simulink model "my_cascade_ramp116_rt"  (R2024a)
settings: Solver=ode3  StartTime=0.0  StopTime=40  FixedStep=0.003  RelTol=1e-3  EnableMultiTasking=on
PreLoadFcn:
  | load('C:\Users\hp\Desktop\group_22\group22_sensor.mat');
undefined symbols (not defined in the file or in its folder): DiscIntNeverNeededParam
libraries: simulink x1
settings Model: SimulationMode=external  Creator=kha  LastModifiedBy=hp
settings SolverCC: AlgebraicLoopSolver=TrustRegion
settings DataIOCC: LimitDataPoints=on  SaveFormat=Array  SignalLoggingSaveFormat=ModelDataLogs  ReturnWorkspaceOutputs=off
settings OptimizationCC: ExpressionDepthLimit=2147483647  InitFltsAndDblsToZero=on  LifeSpan=inf
settings DebuggingCC: SaveWithParameterizedLinksMsg=none  UnderspecifiedInitializationDetection=Classic  MergeDetectMultiDrivingBlocksExec=none  SolverPrmCheckMsg=warning  FcnCallInpInsideContextMsg=warning  UnconnectedInputMsg=warning  UnconnectedOutputMsg=warning  UnconnectedLineMsg=warning  StateNameClashWarn=warning  SFUnexpectedBacktrackingDiag=warning  SFNoUnconditionalDefaultTransitionDiag=warning  SFExecutionAtInitializationDiag=none  ArithmeticOperatorsInVariantConditions=warning
settings HardwareCC: ProdBitPerPointer=32  ProdBitPerSizeT=32  ProdBitPerPtrDiffT=32  ProdLargestAtomicFloat=None  ProdIntDivRoundTo=Undefined  ProdEndianess=Unspecified  ProdWordSize=32  ProdHWDeviceType=32-bit Generic
settings ModelReferenceCC: EnableRefExpFcnMdlSchedulingChecks=on  PropagateSignalLabelsOutOfModel=off
settings SFSimCC: SimUseLocalCustomCode=off  CustomCodeUndefinedFunction=UseInterfaceOnly
settings RTWCC: Description=MLS1EM-RTDAC/USB2 (Visual C/C++)  SystemTargetFile=mls1em_rtcon_usb2.tlc  TemplateMakefile=MLS1EM_RTCON_VC_USB2_x64.tmf  RTWUseLocalCustomCode=off  GPUComputeCapability=3.5  DLArmComputeVersion=19.05
settings CodeAppCC: StateflowObjectComments=on
settings STFCustomTargetCC: TargetLangStandard=C89/C90 (ANSI)  ModelReferenceCompliant=off  CombineOutputUpdateFcns=on  MatFileLogging=on  GRTInterface=off  UseToolchainInfoCompliant=off  SystemTargetFile=mls1em_rtcon_usb2.tlc
settings GRTTargetCC: TargetLangStandard=C89/C90 (ANSI)  ModelReferenceCompliant=off  ParMdlRefBuildCompliant=off  CompOptLevelCompliant=off  ConcurrentExecutionCompliant=off  CPPClassGenCompliant=off  UseToolchainInfoCompliant=off  ExtMode=on  ExtModeMexFile=rtcon_ext_comm
settings ConfigComp: CovMetricSettings=dw  CovSaveCumulativeToWorkspaceVar=on  CovSaveSingleToWorkspaceVar=on  CovExternalEMLEnable=off  CovSFcnEnable=off

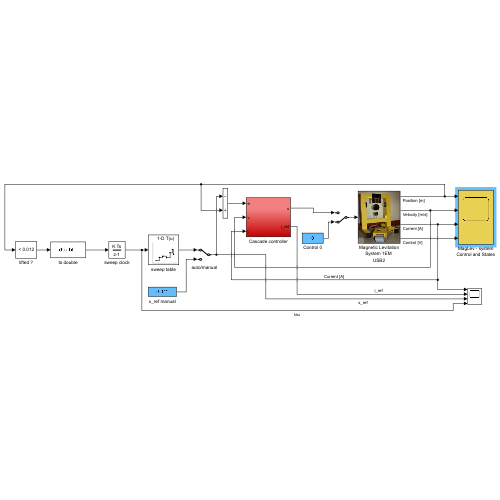
[thumbnail: Simulink's stored preview of the top-level diagram]
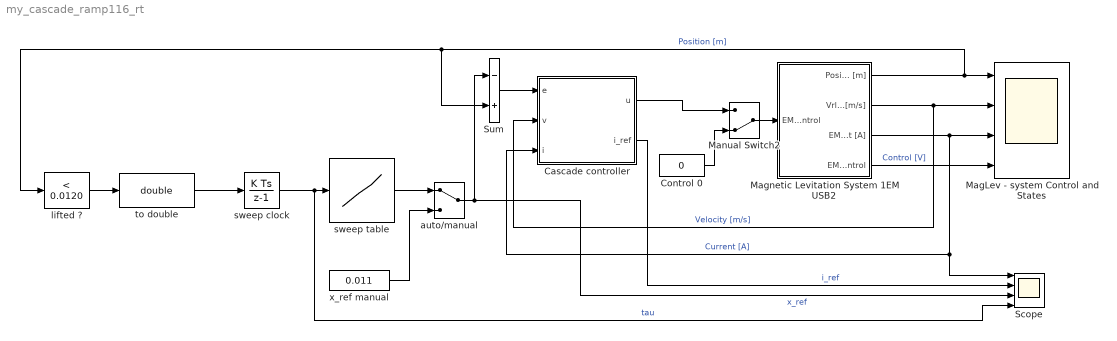
== system my_cascade_ramp116_rt ==
  Cascade controller : Subsystem
  Control 0 : Constant  Value=0
  MagLev - system Control and States : Scope  NumInputPorts=4
  Magnetic Levitation System 1EM USB2 : Subsystem  mask(Magnetic Levitation MLS1EM - System){RTDACUSB2IDX=-1, T0=0.003}
      mask prompts: RTDACUSB2IDX "RT-DAC/USB2 Board Idx (-1) for auto detect"; T0 "Sample time [s]"
      mask help:
      | MagLev MLS2EM - System connection for the real-time operating mode, RT-DAC/USB2 interface
      | (c) InTeCo 2015
      mask Display: image(imread('mls1em_usb2.tiff'));
  Manual Switch2 : ManualSwitch  CurrentSetting=0
  Scope : Scope  NumInputPorts=4
  Sum : Sum  Inputs=-+  InputSameDT=on  SaturateOnIntegerOverflow=on  OutDataTypeStr=Inherit: Same as first input
  auto/manual : ManualSwitch
  lifted ? : simulink/Logic and Bit Operations/Compare To Constant  relop=<  const=0.0120  OutDataTypeStr=boolean
  sweep clock : DiscreteIntegrator  SampleTime=0.003  ICPrevOutput=DiscIntNeverNeededParam  ICPrevScaledInput=DiscIntNeverNeededParam
  sweep table : Lookup_n-D  NumberOfTableDimensions=1  BreakpointsForDimension1=[0 5 10 15.5 21 26]  Table=[11 10.5 10.5 11.6 10.5 10.5]*1e-3  InterpMethod=Flat  InternalRulePriority=Speed  RndMeth=Simplest
  to double : DataTypeConversion  OutDataTypeStr=double  SaturateOnIntegerOverflow=off  RndMeth=Floor
  x_ref manual : Constant  Value=0.011
  wires:
  Control 0/1 -> Manual Switch2/2
  Magnetic Levitation System 1EM USB2/1(Position [m]) -> lifted ?/1, Sum/2, MagLev - system Control and States/1  "Position [m]"
  Magnetic Levitation System 1EM USB2/2(Vrlocity [m/s]) -> Cascade controller/2(v), MagLev - system Control and States/2  "Velocity [m/s]"
  Magnetic Levitation System 1EM USB2/3(EM1 Current [A]) -> Scope/1, Cascade controller/3(i), MagLev - system Control and States/3  "Current [A]"
  Magnetic Levitation System 1EM USB2/4(EM1 control) -> MagLev - system Control and States/4  "Control [V]"
  Manual Switch2/1 -> Magnetic Levitation System 1EM USB2/1(EM1 Control)
  Sum/1 -> Cascade controller/1(e)
  Cascade controller/1(u) -> Manual Switch2/1
  Cascade controller/2(i_ref) -> Scope/2  "i_ref"
  lifted ?/1 -> to double/1
  to double/1 -> sweep clock/1
  sweep clock/1 -> Scope/4, sweep table/1  "tau"
  sweep table/1 -> auto/manual/1
  x_ref manual/1 -> auto/manual/2
  auto/manual/1 -> Scope/3, Sum/1  "x_ref"

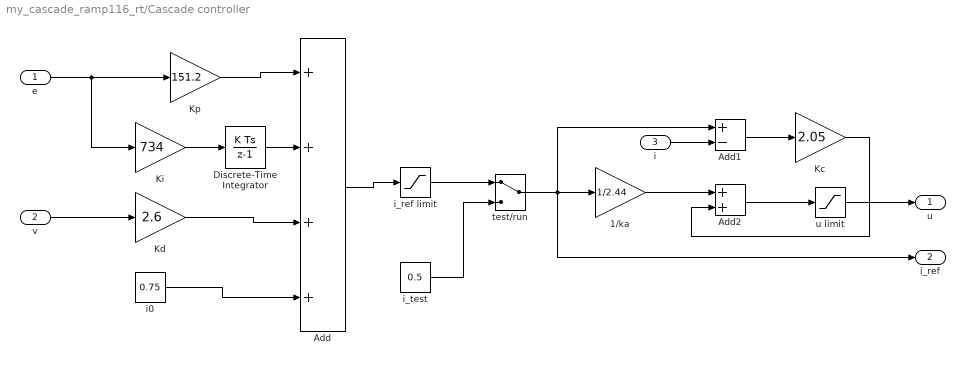
== system my_cascade_ramp116_rt/Cascade controller ==
  e : Inport
  v : Inport  Port=2
  i : Inport  Port=3
  1/ka : Gain  Gain=1/2.44
  Add : Sum  Inputs=++++
  Add1 : Sum  Inputs=+-
  Add2 : Sum
  Discrete-Time Integrator : DiscreteIntegrator  SampleTime=0.003  LimitOutput=on  UpperSaturationLimit=0.3  LowerSaturationLimit=-0.3  ICPrevOutput=DiscIntNeverNeededParam  ICPrevScaledInput=DiscIntNeverNeededParam
  Kc : Gain  Gain=2.05
  Kd : Gain  Gain=2.6
  Ki : Gain  Gain=734
  Kp : Gain  Gain=151.2
  i0 : Constant  Value=0.75
  i_ref limit : Saturate  UpperLimit=2.0  LowerLimit=0
      settings: AttributesFormatString=|
      | UL: %<UpperLimit>
      | LL: %<LowerLimit>
  i_test : Constant  Value=0.5
  test/run : ManualSwitch
  u limit : Saturate  UpperLimit=0.9  LowerLimit=0
      settings: AttributesFormatString=|
      | UL: %<UpperLimit>
      | LL: %<LowerLimit>
  u : Outport
  i_ref : Outport  Port=2
  wires:
  e/1 -> Kp/1, Ki/1
  Kp/1 -> Add/1
  Ki/1 -> Discrete-Time Integrator/1
  Discrete-Time Integrator/1 -> Add/2
  Kd/1 -> Add/3
  v/1 -> Kd/1
  i0/1 -> Add/4
  Add/1 -> i_ref limit/1
  i_ref limit/1 -> test/run/1
  i_test/1 -> test/run/2
  test/run/1 -> i_ref/1, 1/ka/1, Add1/1
  1/ka/1 -> Add2/1
  i/1 -> Add1/2
  Add1/1 -> Kc/1
  Kc/1 -> Add2/2
  Add2/1 -> u limit/1
  u limit/1 -> u/1

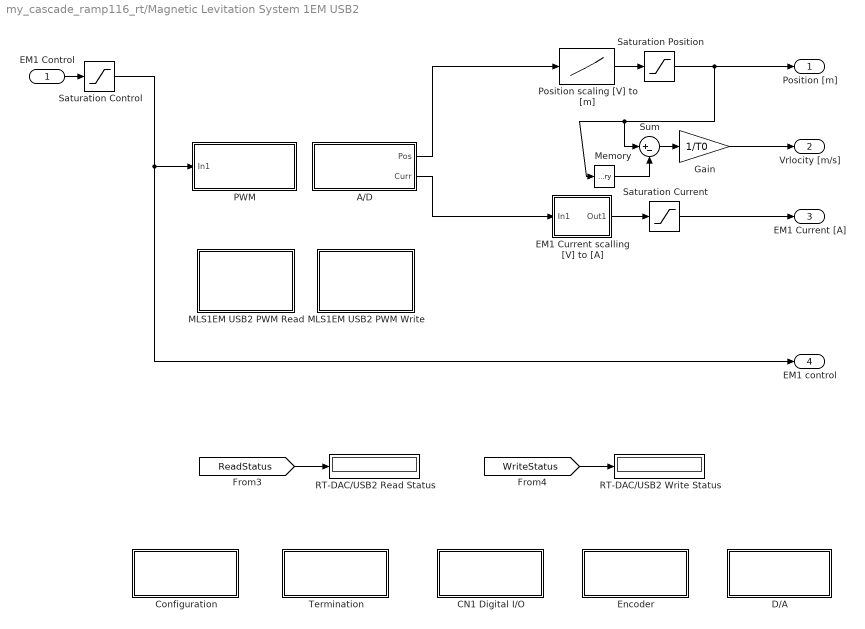
== system my_cascade_ramp116_rt/Magnetic Levitation System 1EM USB2 ==
  EM1 Control : Inport
  A/D : Subsystem
      mask Display: disp('A / D')
  CN1 Digital I/O : Subsystem
      mask Display: disp('CN1 Digital I/O')
  Configuration : Subsystem
      mask Display: disp('CONFIGURATION')
  D/A : Subsystem
      mask Display: disp('D / A')
  EM1 Current scalling [V] to [A] : Subsystem
      mask Display: plot([0    0.5000    1.0000    1.5000    2.0000    2.5000], [-0.0317    0.4951    1.0302    1.5738    2.1258    2.6863]);
  Encoder : Subsystem
      mask Display: disp('Encoder')
  Gain : Gain  Gain=1/T0
  MLS1EM USB2 PWM Read : Subsystem
      mask Display: disp( 'RT-DAC/USB2' )
  MLS1EM USB2 PWM Write : Subsystem
      mask Display: disp( 'RT-DAC/USB2')
  Memory : Memory
  PWM : Subsystem
      mask Display: disp('PWM')
  Position scaling [V] to [m] : Lookup  InputValues=SensorData.Sensor_V(end:-1:1)  Table=SensorData.Distance_m(end:-1:1)
  RT-DAC/USB2 Read Status : Display
  RT-DAC/USB2 Write Status : Display
  Saturation Control : Saturate  UpperLimit=5  LowerLimit=0
  Saturation Current : Saturate  UpperLimit=30  LowerLimit=-30
  Saturation Position : Saturate  UpperLimit=0.02  LowerLimit=0
  Sum : Sum  Inputs=|+-
  Termination : Subsystem
      mask Display: disp('CONFIGURATION')
  Position [m] : Outport  VectorParamsAs1DForOutWhenUnconnected=off
  Vrlocity [m/s] : Outport  Port=2  VectorParamsAs1DForOutWhenUnconnected=off
  EM1 Current [A] : Outport  Port=3  VectorParamsAs1DForOutWhenUnconnected=off
  EM1 control : Outport  Port=4  VectorParamsAs1DForOutWhenUnconnected=off
  wires:
  EM1 Control/1 -> Saturation Control/1
  Saturation Position/1 -> Position [m]/1, Sum/1, Memory/1
  Gain/1 -> Vrlocity [m/s]/1
  Saturation Control/1 -> PWM/1(In1), EM1 control/1
  Memory/1 -> Sum/2
  Position scaling [V] to [m]/1 -> Saturation Position/1
  Sum/1 -> Gain/1
  EM1 Current scalling [V] to [A]/1(Out1) -> Saturation Current/1
  [ReadStatus] -> RT-DAC/USB2 Read Status/1
  [WriteStatus] -> RT-DAC/USB2 Write Status/1
  A/D/1(Pos) -> Position scaling [V] to [m]/1
  A/D/2(Curr) -> EM1 Current scalling [V] to [A]/1(In1)
  Saturation Current/1 -> EM1 Current [A]/1

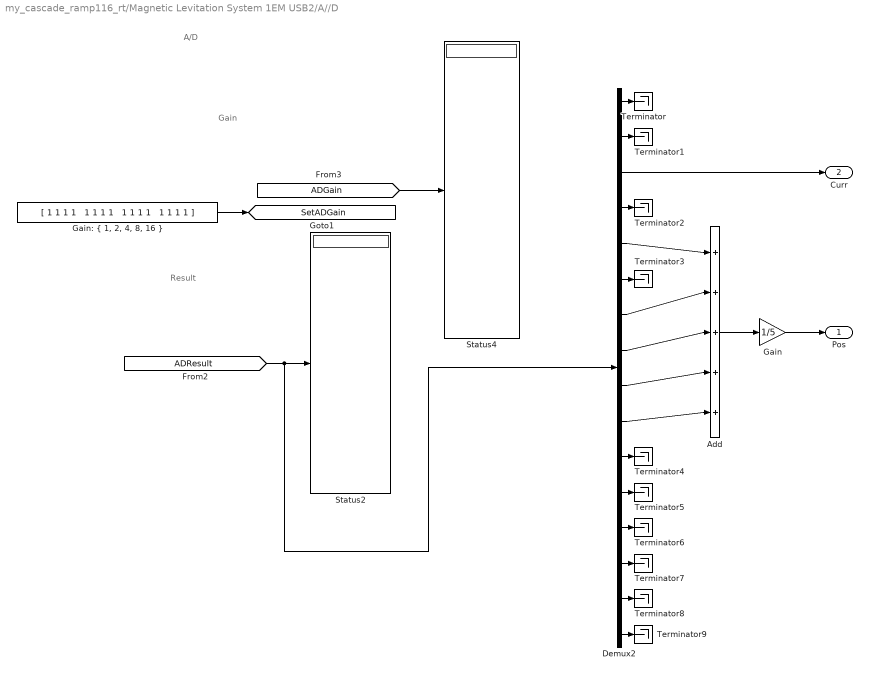
== system my_cascade_ramp116_rt/Magnetic Levitation System 1EM USB2/A//D ==
  note: A/D
  note: Gain
  note: Result
  Add : Sum  Inputs=+|++++
  Demux2 : Demux  Outputs=16
      settings: DisplayOption=none
  Gain : Gain  Gain=1/5
  "Gain: { 1, 2, 4, 8, 16 }" : Constant  Value="[ 1 1 1 1   1 1 1 1   1 1 1 1   1 1 1 1 ]"
  Status2 : Display
  Status4 : Display
  Terminator{,1..9} (10 alike) : Terminator
  Pos : Outport  VectorParamsAs1DForOutWhenUnconnected=off
  Curr : Outport  Port=2  VectorParamsAs1DForOutWhenUnconnected=off
  tag scope: SetADGain=global
  wires:
  [ADResult] -> Demux2/1, Status2/1
  [ADGain] -> Status4/1
  "Gain: { 1, 2, 4, 8, 16 }"/1 -> [SetADGain]
  Add/1 -> Gain/1
  Gain/1 -> Pos/1
  Demux2/3 -> Curr/1
  Demux2/5 -> Add/1
  Demux2/7 -> Add/2
  Demux2/8 -> Add/3
  Demux2/9 -> Add/4
  Demux2/10 -> Add/5
  Demux2/1 -> Terminator/1
  Demux2/2 -> Terminator1/1
  Demux2/4 -> Terminator2/1
  Demux2/6 -> Terminator3/1
  Demux2/11 -> Terminator4/1
  Demux2/12 -> Terminator5/1
  Demux2/13 -> Terminator6/1
  Demux2/14 -> Terminator7/1
  Demux2/15 -> Terminator8/1
  Demux2/16 -> Terminator9/1

== system my_cascade_ramp116_rt/Magnetic Levitation System 1EM USB2/CN1 Digital I//O ==
  note: Digital I/Os
  note: Pin mode
  note: Direction
  note: Output
  note: Input
  Data Type Conversion1 : DataTypeConversion  OutDataTypeStr=uint32  SaturateOnIntegerOverflow=off  RndMeth=Floor
  Data Type Conversion2 : DataTypeConversion  OutDataTypeStr=int32  SaturateOnIntegerOverflow=off  RndMeth=Floor
  Data Type Conversion3 : DataTypeConversion  OutDataTypeStr=uint32  SaturateOnIntegerOverflow=off  RndMeth=Floor
  Data Type Conversion4 : DataTypeConversion  OutDataTypeStr=int32  SaturateOnIntegerOverflow=off  RndMeth=Floor
  Status{1..4} (4 alike) : Display
      settings: Format=hex (Stored Integer)
  Subsystem : Subsystem
      mask Display: disp( 'CN1 Direction' )
  Subsystem1 : Subsystem
      mask Display: disp( 'CN1 Output' )
  Subsystem2 : Subsystem
      mask Display: disp( 'CN1 Pin Mode' )
  wires:
  Data Type Conversion1/1 -> Status1/1
  Data Type Conversion2/1 -> Status3/1
  [CN1Direction] -> Data Type Conversion1/1
  [CN1PinMode] -> Data Type Conversion2/1
  Data Type Conversion3/1 -> Status2/1
  Data Type Conversion4/1 -> Status4/1
  [CN1Output] -> Data Type Conversion4/1
  [CN1Input] -> Data Type Conversion3/1

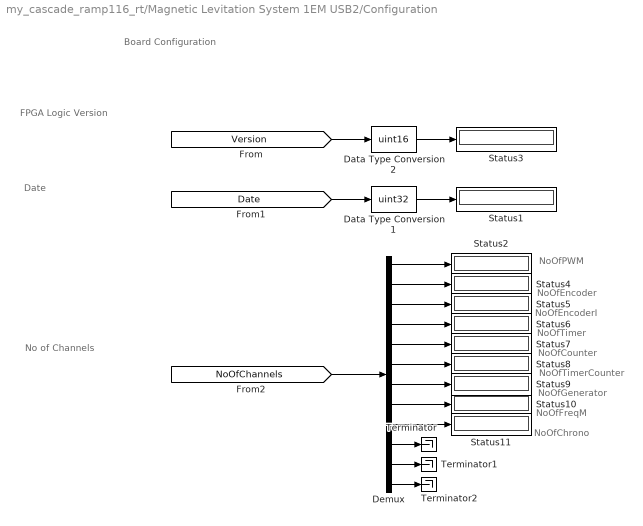
== system my_cascade_ramp116_rt/Magnetic Levitation System 1EM USB2/Configuration ==
  note: NoOfPWM
  note: NoOfEncoder
  note: NoOfEncoderI
  note: NoOfTimer
  note: NoOfCounter
  note: NoOfTimerCounter
  note: NoOfGenerator
  note: NoOfFreqM
  note: NoOfChrono
  note: Board Configuration
  note: FPGA Logic
      | Version
  note: Date
  note: No of
      | Channels
  Data Type Conversion1 : DataTypeConversion  OutDataTypeStr=uint32  SaturateOnIntegerOverflow=off  RndMeth=Floor
  Data Type Conversion2 : DataTypeConversion  OutDataTypeStr=uint16  SaturateOnIntegerOverflow=off  RndMeth=Floor
  Demux : Demux  Outputs=12
  Status{1..11} (11 alike) : Display
      Status1 settings: Format=hex (Stored Integer)
      Status3 settings: Format=hex (Stored Integer)
  Terminator : Terminator
  Terminator1 : Terminator
  Terminator2 : Terminator
  wires:
  [Version] -> Data Type Conversion2/1
  [Date] -> Data Type Conversion1/1
  Data Type Conversion2/1 -> Status3/1
  Data Type Conversion1/1 -> Status1/1
  [NoOfChannels] -> Demux/1
  Demux/1 -> Status2/1
  Demux/2 -> Status4/1
  Demux/3 -> Status5/1
  Demux/4 -> Status6/1
  Demux/5 -> Status7/1
  Demux/6 -> Status8/1
  Demux/7 -> Status9/1
  Demux/8 -> Status10/1
  Demux/9 -> Status11/1
  Demux/10 -> Terminator/1
  Demux/11 -> Terminator1/1
  Demux/12 -> Terminator2/1

== system my_cascade_ramp116_rt/Magnetic Levitation System 1EM USB2/D//A ==
  note: D/A
  note: D/A outputs range: -10.0 - +10.0
  D/A {0..3} (4 alike) : Constant  Value=0
  Mux1 : Mux
  Status4 : Display
  tag scope: SetDA=global
  wires:
  Mux1/1 -> [SetDA]
  [DA] -> Status4/1
  D/A 1/1 -> Mux1/2
  D/A 2/1 -> Mux1/3
  D/A 3/1 -> Mux1/4
  D/A 0/1 -> Mux1/1

== system my_cascade_ramp116_rt/Magnetic Levitation System 1EM USB2/EM1 Current scalling [V] to [A] ==
  In1 : Inport
  Fcn : Fcn  Expr=0.598941443808775*u(1)-0.017342099593970
  Out1 : Outport  VectorParamsAs1DForOutWhenUnconnected=off
  wires:
  In1/1 -> Fcn/1
  Fcn/1 -> Out1/1

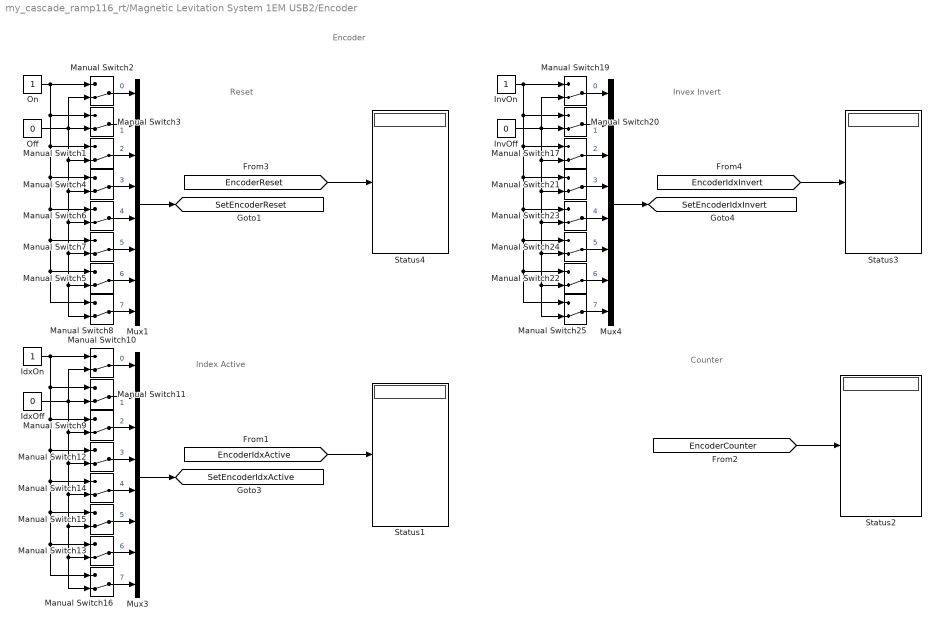
== system my_cascade_ramp116_rt/Magnetic Levitation System 1EM USB2/Encoder ==
  note: Counter
  note: Reset
  note: Encoder
  note: Index Active
  note: Invex Invert
  IdxOff : Constant  Value=0
  IdxOn : Constant
  InvOff : Constant  Value=0
  InvOn : Constant
  Manual Switch{1..17,19..25} (24 alike) : ManualSwitch  CurrentSetting=0
  Mux1 : Mux  Inputs=8
  Mux3 : Mux  Inputs=8
  Mux4 : Mux  Inputs=8
  Off : Constant  Value=0
  On : Constant
  Status{1..4} (4 alike) : Display
  tag scope: SetEncoderIdxActive=global, SetEncoderIdxInvert=global, SetEncoderReset=global
  wires:
  Manual Switch8/1 -> Mux1/8  "7"
  Manual Switch5/1 -> Mux1/7  "6"
  Manual Switch1/1 -> Mux1/3  "2"
  Manual Switch4/1 -> Mux1/4  "3"
  Manual Switch7/1 -> Mux1/6  "5"
  Manual Switch6/1 -> Mux1/5  "4"
  Manual Switch3/1 -> Mux1/2  "1"
  Manual Switch2/1 -> Mux1/1  "0"
  Off/1 -> Manual Switch8/2, Manual Switch5/2, Manual Switch7/2, Manual Switch6/2, Manual Switch4/2, Manual Switch1/2, Manual Switch2/2, Manual Switch3/2
  On/1 -> Manual Switch1/1, Manual Switch4/1, Manual Switch6/1, Manual Switch7/1, Manual Switch5/1, Manual Switch8/1, Manual Switch3/1, Manual Switch2/1
  Mux1/1 -> [SetEncoderReset]
  [EncoderReset] -> Status4/1
  [EncoderCounter] -> Status2/1
  Manual Switch16/1 -> Mux3/8  "7"
  Manual Switch13/1 -> Mux3/7  "6"
  Manual Switch9/1 -> Mux3/3  "2"
  Manual Switch12/1 -> Mux3/4  "3"
  Manual Switch15/1 -> Mux3/6  "5"
  Manual Switch14/1 -> Mux3/5  "4"
  Manual Switch11/1 -> Mux3/2  "1"
  Manual Switch10/1 -> Mux3/1  "0"
  IdxOff/1 -> Manual Switch11/2, Manual Switch10/2, Manual Switch9/2, Manual Switch12/2, Manual Switch14/2, Manual Switch15/2, Manual Switch13/2, Manual Switch16/2
  IdxOn/1 -> Manual Switch10/1, Manual Switch11/1, Manual Switch16/1, Manual Switch13/1, Manual Switch15/1, Manual Switch14/1, Manual Switch12/1, Manual Switch9/1
  Mux3/1 -> [SetEncoderIdxActive]
  [EncoderIdxActive] -> Status1/1
  Manual Switch25/1 -> Mux4/8  "7"
  Manual Switch22/1 -> Mux4/7  "6"
  Manual Switch17/1 -> Mux4/3  "2"
  Manual Switch21/1 -> Mux4/4  "3"
  Manual Switch24/1 -> Mux4/6  "5"
  Manual Switch23/1 -> Mux4/5  "4"
  Manual Switch20/1 -> Mux4/2  "1"
  Manual Switch19/1 -> Mux4/1  "0"
  InvOff/1 -> Manual Switch25/2, Manual Switch22/2, Manual Switch24/2, Manual Switch23/2, Manual Switch21/2, Manual Switch17/2, Manual Switch19/2, Manual Switch20/2
  InvOn/1 -> Manual Switch17/1, Manual Switch21/1, Manual Switch23/1, Manual Switch24/1, Manual Switch22/1, Manual Switch25/1, Manual Switch20/1, Manual Switch19/1
  Mux4/1 -> [SetEncoderIdxInvert]
  [EncoderIdxInvert] -> Status3/1

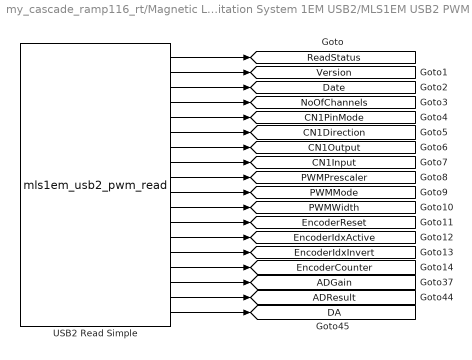
== system my_cascade_ramp116_rt/Magnetic Levitation System 1EM USB2/MLS1EM USB2 PWM Read ==
  USB2 Read Simple : S-Function  FunctionName=mls1em_usb2_pwm_read  Parameters=-1, T0  SFunctionDeploymentMode=off  EnableBusSupport=off
  tag scope: ADGain=global, ADResult=global, CN1Direction=global, CN1Input=global, CN1Output=global, CN1PinMode=global, DA=global, Date=global, EncoderCounter=global, EncoderIdxActive=global, EncoderIdxInvert=global, EncoderReset=global, NoOfChannels=global, PWMMode=global, PWMPrescaler=global, PWMWidth=global, ReadStatus=global, Version=global
  wires:
  USB2 Read Simple/18 -> [DA]
  USB2 Read Simple/17 -> [ADResult]
  USB2 Read Simple/16 -> [ADGain]
  USB2 Read Simple/1 -> [ReadStatus]
  USB2 Read Simple/2 -> [Version]
  USB2 Read Simple/3 -> [Date]
  USB2 Read Simple/4 -> [NoOfChannels]
  USB2 Read Simple/5 -> [CN1PinMode]
  USB2 Read Simple/6 -> [CN1Direction]
  USB2 Read Simple/7 -> [CN1Output]
  USB2 Read Simple/8 -> [CN1Input]
  USB2 Read Simple/9 -> [PWMPrescaler]
  USB2 Read Simple/11 -> [PWMWidth]
  USB2 Read Simple/10 -> [PWMMode]
  USB2 Read Simple/12 -> [EncoderReset]
  USB2 Read Simple/13 -> [EncoderIdxActive]
  USB2 Read Simple/14 -> [EncoderIdxInvert]
  USB2 Read Simple/15 -> [EncoderCounter]

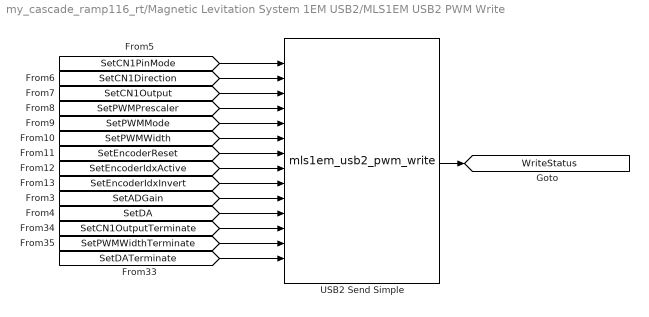
== system my_cascade_ramp116_rt/Magnetic Levitation System 1EM USB2/MLS1EM USB2 PWM Write ==
  USB2 Send Simple : S-Function  FunctionName=mls1em_usb2_pwm_write  Parameters=-1, T0  SFunctionDeploymentMode=off  EnableBusSupport=off
  tag scope: WriteStatus=global
  wires:
  [SetEncoderIdxInvert] -> USB2 Send Simple/9
  [SetPWMWidthTerminate] -> USB2 Send Simple/13
  [SetCN1OutputTerminate] -> USB2 Send Simple/12
  [SetDATerminate] -> USB2 Send Simple/14
  [SetDA] -> USB2 Send Simple/11
  [SetADGain] -> USB2 Send Simple/10
  [SetEncoderIdxActive] -> USB2 Send Simple/8
  [SetEncoderReset] -> USB2 Send Simple/7
  [SetPWMWidth] -> USB2 Send Simple/6
  [SetPWMMode] -> USB2 Send Simple/5
  [SetPWMPrescaler] -> USB2 Send Simple/4
  [SetCN1Output] -> USB2 Send Simple/3
  [SetCN1Direction] -> USB2 Send Simple/2
  [SetCN1PinMode] -> USB2 Send Simple/1
  USB2 Send Simple/1 -> [WriteStatus]

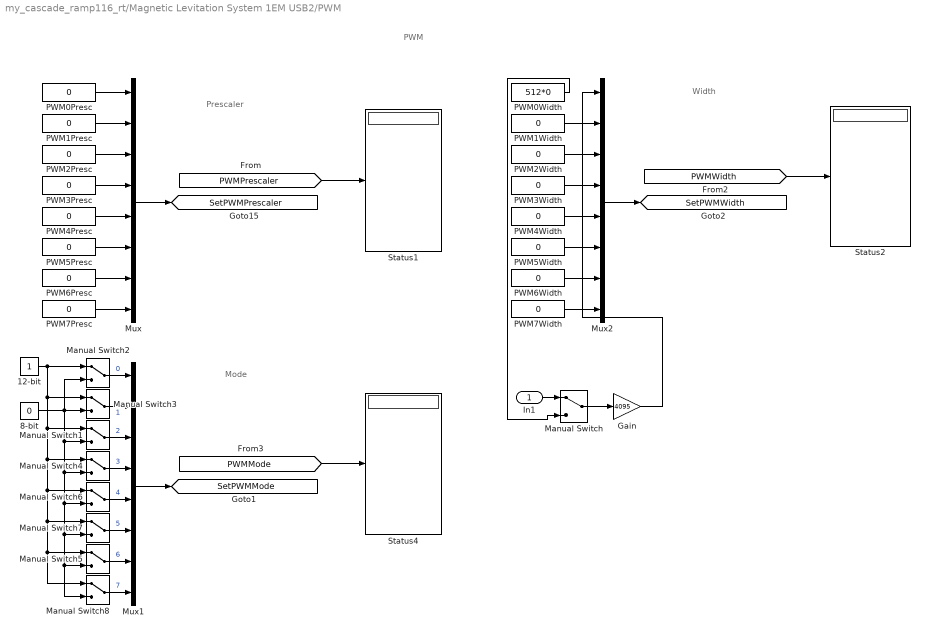
== system my_cascade_ramp116_rt/Magnetic Levitation System 1EM USB2/PWM ==
  note: PWM
  note: Prescaler
  note: Mode
  note: Width
  In1 : Inport
  12-bit : Constant
  8-bit : Constant  Value=0
  Gain : Gain  Gain=4095
  Manual Switch{,1..8} (9 alike) : ManualSwitch
  Mux : Mux  Inputs=8
  Mux1 : Mux  Inputs=8
  Mux2 : Mux  Inputs=8
  PWM0Presc : Constant  Value=0
  PWM0Width : Constant  Value=512*0
  PWM1Presc : Constant  Value=0
  PWM1Width : Constant  Value=0
  PWM2Presc : Constant  Value=0
  PWM2Width : Constant  Value=0
  PWM3Presc : Constant  Value=0
  PWM3Width : Constant  Value=0
  PWM4Presc : Constant  Value=0
  PWM4Width : Constant  Value=0
  PWM5Presc : Constant  Value=0
  PWM5Width : Constant  Value=0
  PWM6Presc : Constant  Value=0
  PWM6Width : Constant  Value=0
  PWM7Presc : Constant  Value=0
  PWM7Width : Constant  Value=0
  Status1 : Display
  Status2 : Display
  Status4 : Display
  tag scope: SetPWMMode=global, SetPWMPrescaler=global, SetPWMWidth=global
  wires:
  Gain/1 -> Mux2/1
  Manual Switch/1 -> Gain/1
  PWM0Width/1 -> Manual Switch/2
  In1/1 -> Manual Switch/1
  [PWMPrescaler] -> Status1/1
  [PWMWidth] -> Status2/1
  PWM0Presc/1 -> Mux/1
  PWM1Presc/1 -> Mux/2
  PWM2Presc/1 -> Mux/3
  PWM3Presc/1 -> Mux/4
  PWM4Presc/1 -> Mux/5
  PWM5Presc/1 -> Mux/6
  PWM6Presc/1 -> Mux/7
  PWM7Presc/1 -> Mux/8
  Mux/1 -> [SetPWMPrescaler]
  [PWMMode] -> Status4/1
  Mux1/1 -> [SetPWMMode]
  PWM2Width/1 -> Mux2/3
  PWM3Width/1 -> Mux2/4
  PWM4Width/1 -> Mux2/5
  PWM5Width/1 -> Mux2/6
  PWM6Width/1 -> Mux2/7
  PWM7Width/1 -> Mux2/8
  Mux2/1 -> [SetPWMWidth]
  12-bit/1 -> Manual Switch2/1, Manual Switch3/1, Manual Switch8/1, Manual Switch5/1, Manual Switch7/1, Manual Switch6/1, Manual Switch4/1, Manual Switch1/1
  8-bit/1 -> Manual Switch3/2, Manual Switch2/2, Manual Switch1/2, Manual Switch4/2, Manual Switch6/2, Manual Switch7/2, Manual Switch5/2, Manual Switch8/2
  Manual Switch2/1 -> Mux1/1  "0"
  Manual Switch3/1 -> Mux1/2  "1"
  Manual Switch6/1 -> Mux1/5  "4"
  Manual Switch7/1 -> Mux1/6  "5"
  Manual Switch4/1 -> Mux1/4  "3"
  Manual Switch1/1 -> Mux1/3  "2"
  Manual Switch5/1 -> Mux1/7  "6"
  Manual Switch8/1 -> Mux1/8  "7"
  PWM1Width/1 -> Mux2/2

== system my_cascade_ramp116_rt/Magnetic Levitation System 1EM USB2/Termination ==
  note: Outputs at termination
  CN1Termination : Constant  Value=0
  DA Termination : Constant  Value=[ 0 0 0 0 ]
  PWMTermination : Constant  Value=[ 0 0 0 0 0 0 0 0 ]
  tag scope: SetCN1OutputTerminate=global, SetDATerminate=global, SetPWMWidthTerminate=global
  wires:
  CN1Termination/1 -> [SetCN1OutputTerminate]
  PWMTermination/1 -> [SetPWMWidthTerminate]
  DA Termination/1 -> [SetDATerminate]

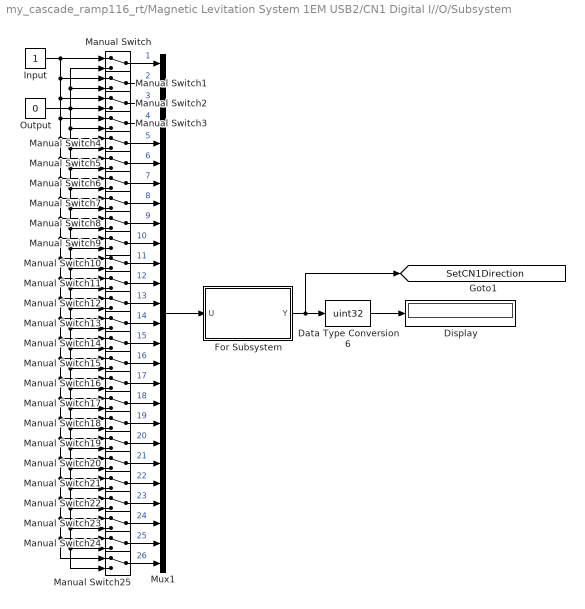
== system my_cascade_ramp116_rt/Magnetic Levitation System 1EM USB2/CN1 Digital I//O/Subsystem ==
  Data Type Conversion6 : DataTypeConversion  OutDataTypeStr=uint32  SaturateOnIntegerOverflow=off  RndMeth=Floor
  Display : Display
      settings: Format=hex (Stored Integer)
  For Subsystem : Subsystem  TreatAsAtomicUnit=on
  Input : Constant
  Manual Switch{,1..25} (26 alike) : ManualSwitch
  Mux1 : Mux  Inputs=26
  Output : Constant  Value=0
  tag scope: SetCN1Direction=global
  wires:
  Input/1 -> Manual Switch/1, Manual Switch1/1, Manual Switch2/1, Manual Switch3/1, Manual Switch4/1, Manual Switch5/1, Manual Switch6/1, Manual Switch7/1, Manual Switch8/1, Manual Switch9/1, Manual Switch10/1, Manual Switch11/1, Manual Switch12/1, Manual Switch13/1, Manual Switch14/1, Manual Switch15/1, Manual Switch16/1, Manual Switch17/1, Manual Switch18/1, Manual Switch19/1, Manual Switch20/1, Manual Switch21/1, Manual Switch22/1, Manual Switch23/1, Manual Switch25/1, Manual Switch24/1
  Output/1 -> Manual Switch/2, Manual Switch1/2, Manual Switch2/2, Manual Switch3/2, Manual Switch4/2, Manual Switch5/2, Manual Switch6/2, Manual Switch7/2, Manual Switch8/2, Manual Switch9/2, Manual Switch10/2, Manual Switch11/2, Manual Switch12/2, Manual Switch13/2, Manual Switch14/2, Manual Switch15/2, Manual Switch16/2, Manual Switch17/2, Manual Switch18/2, Manual Switch19/2, Manual Switch20/2, Manual Switch21/2, Manual Switch22/2, Manual Switch23/2, Manual Switch25/2, Manual Switch24/2
  Manual Switch/1 -> Mux1/1  "1"
  Manual Switch1/1 -> Mux1/2  "2"
  Manual Switch2/1 -> Mux1/3  "3"
  Manual Switch3/1 -> Mux1/4  "4"
  Manual Switch4/1 -> Mux1/5  "5"
  Manual Switch5/1 -> Mux1/6  "6"
  Manual Switch6/1 -> Mux1/7  "7"
  Manual Switch7/1 -> Mux1/8  "8"
  Manual Switch8/1 -> Mux1/9  "9"
  Manual Switch9/1 -> Mux1/10  "10"
  Manual Switch10/1 -> Mux1/11  "11"
  Manual Switch11/1 -> Mux1/12  "12"
  Manual Switch12/1 -> Mux1/13  "13"
  Manual Switch13/1 -> Mux1/14  "14"
  Manual Switch14/1 -> Mux1/15  "15"
  Manual Switch15/1 -> Mux1/16  "16"
  Manual Switch16/1 -> Mux1/17  "17"
  Manual Switch17/1 -> Mux1/18  "18"
  Manual Switch18/1 -> Mux1/19  "19"
  Manual Switch19/1 -> Mux1/20  "20"
  Manual Switch20/1 -> Mux1/21  "21"
  Manual Switch21/1 -> Mux1/22  "22"
  Manual Switch22/1 -> Mux1/23  "23"
  Manual Switch23/1 -> Mux1/24  "24"
  Manual Switch24/1 -> Mux1/25  "25"
  Manual Switch25/1 -> Mux1/26  "26"
  Mux1/1 -> For Subsystem/1(U)
  For Subsystem/1(Y) -> Data Type Conversion6/1, [SetCN1Direction]
  Data Type Conversion6/1 -> Display/1

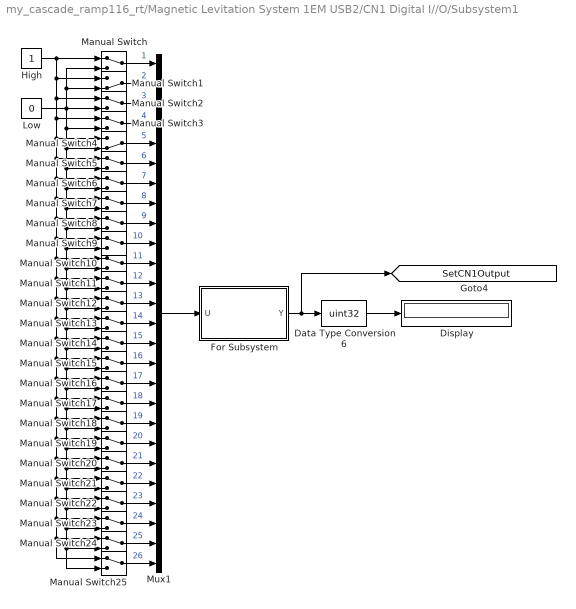
== system my_cascade_ramp116_rt/Magnetic Levitation System 1EM USB2/CN1 Digital I//O/Subsystem1 ==
  Data Type Conversion6 : DataTypeConversion  OutDataTypeStr=uint32  SaturateOnIntegerOverflow=off  RndMeth=Floor
  Display : Display
      settings: Format=hex (Stored Integer)
  For Subsystem : Subsystem  TreatAsAtomicUnit=on
  High : Constant
  Low : Constant  Value=0
  Manual Switch{,2..3,5..25} (24 alike) : ManualSwitch
  Manual Switch1 : ManualSwitch  CurrentSetting=0
  Manual Switch4 : ManualSwitch  CurrentSetting=0
  Mux1 : Mux  Inputs=26
  tag scope: SetCN1Output=global
  wires:
  Data Type Conversion6/1 -> Display/1
  For Subsystem/1(Y) -> Data Type Conversion6/1, [SetCN1Output]
  Mux1/1 -> For Subsystem/1(U)
  Manual Switch25/1 -> Mux1/26  "26"
  Manual Switch24/1 -> Mux1/25  "25"
  Manual Switch23/1 -> Mux1/24  "24"
  Manual Switch22/1 -> Mux1/23  "23"
  Manual Switch21/1 -> Mux1/22  "22"
  Manual Switch20/1 -> Mux1/21  "21"
  Manual Switch19/1 -> Mux1/20  "20"
  Manual Switch18/1 -> Mux1/19  "19"
  Manual Switch17/1 -> Mux1/18  "18"
  Manual Switch16/1 -> Mux1/17  "17"
  Manual Switch15/1 -> Mux1/16  "16"
  Manual Switch14/1 -> Mux1/15  "15"
  Manual Switch13/1 -> Mux1/14  "14"
  Manual Switch12/1 -> Mux1/13  "13"
  Manual Switch11/1 -> Mux1/12  "12"
  Manual Switch10/1 -> Mux1/11  "11"
  Manual Switch9/1 -> Mux1/10  "10"
  Manual Switch8/1 -> Mux1/9  "9"
  Manual Switch7/1 -> Mux1/8  "8"
  Manual Switch6/1 -> Mux1/7  "7"
  Manual Switch5/1 -> Mux1/6  "6"
  Manual Switch4/1 -> Mux1/5  "5"
  Manual Switch3/1 -> Mux1/4  "4"
  Manual Switch2/1 -> Mux1/3  "3"
  Manual Switch1/1 -> Mux1/2  "2"
  Manual Switch/1 -> Mux1/1  "1"
  Low/1 -> Manual Switch24/2, Manual Switch25/2, Manual Switch23/2, Manual Switch22/2, Manual Switch21/2, Manual Switch20/2, Manual Switch19/2, Manual Switch18/2, Manual Switch17/2, Manual Switch16/2, Manual Switch15/2, Manual Switch14/2, Manual Switch13/2, Manual Switch12/2, Manual Switch11/2, Manual Switch10/2, Manual Switch9/2, Manual Switch8/2, Manual Switch7/2, Manual Switch6/2, Manual Switch5/2, Manual Switch4/2, Manual Switch3/2, Manual Switch2/2, Manual Switch1/2, Manual Switch/2
  High/1 -> Manual Switch24/1, Manual Switch25/1, Manual Switch23/1, Manual Switch22/1, Manual Switch21/1, Manual Switch20/1, Manual Switch19/1, Manual Switch18/1, Manual Switch17/1, Manual Switch16/1, Manual Switch15/1, Manual Switch14/1, Manual Switch13/1, Manual Switch12/1, Manual Switch11/1, Manual Switch10/1, Manual Switch9/1, Manual Switch8/1, Manual Switch7/1, Manual Switch6/1, Manual Switch5/1, Manual Switch4/1, Manual Switch3/1, Manual Switch2/1, Manual Switch1/1, Manual Switch/1

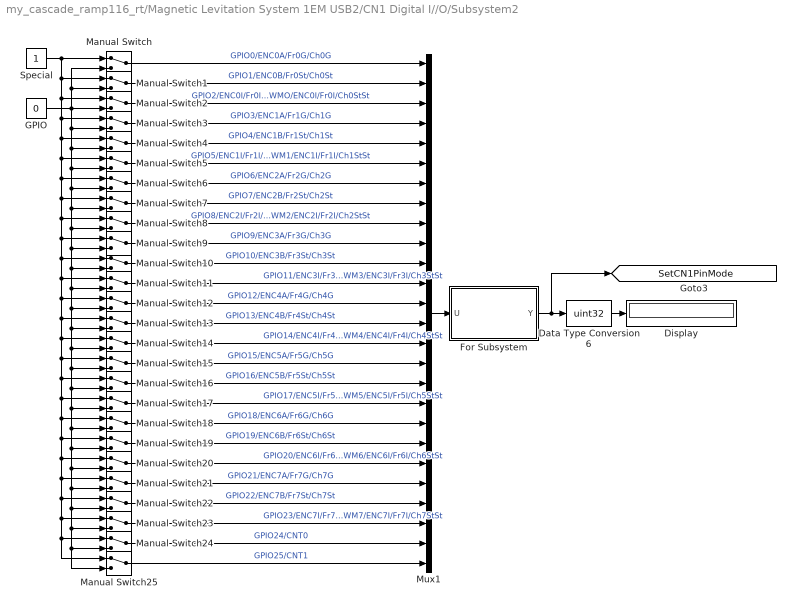
== system my_cascade_ramp116_rt/Magnetic Levitation System 1EM USB2/CN1 Digital I//O/Subsystem2 ==
  Data Type Conversion6 : DataTypeConversion  OutDataTypeStr=uint32  SaturateOnIntegerOverflow=off  RndMeth=Floor
  Display : Display
      settings: Format=hex (Stored Integer)
  For Subsystem : Subsystem  TreatAsAtomicUnit=on
  GPIO : Constant  Value=0
  Manual Switch{,1..25} (26 alike) : ManualSwitch
  Mux1 : Mux  Inputs=26
  Special : Constant
  tag scope: SetCN1PinMode=global
  wires:
  Special/1 -> Manual Switch/1, Manual Switch1/1, Manual Switch2/1, Manual Switch3/1, Manual Switch4/1, Manual Switch5/1, Manual Switch6/1, Manual Switch7/1, Manual Switch8/1, Manual Switch9/1, Manual Switch10/1, Manual Switch11/1, Manual Switch12/1, Manual Switch13/1, Manual Switch14/1, Manual Switch15/1, Manual Switch16/1, Manual Switch17/1, Manual Switch18/1, Manual Switch19/1, Manual Switch20/1, Manual Switch21/1, Manual Switch22/1, Manual Switch23/1, Manual Switch25/1, Manual Switch24/1
  GPIO/1 -> Manual Switch/2, Manual Switch1/2, Manual Switch2/2, Manual Switch3/2, Manual Switch4/2, Manual Switch5/2, Manual Switch6/2, Manual Switch7/2, Manual Switch8/2, Manual Switch9/2, Manual Switch10/2, Manual Switch11/2, Manual Switch12/2, Manual Switch13/2, Manual Switch14/2, Manual Switch15/2, Manual Switch16/2, Manual Switch17/2, Manual Switch18/2, Manual Switch19/2, Manual Switch20/2, Manual Switch21/2, Manual Switch22/2, Manual Switch23/2, Manual Switch25/2, Manual Switch24/2
  Manual Switch/1 -> Mux1/1  "GPIO0/ENC0A/Fr0G/Ch0G"
  Manual Switch1/1 -> Mux1/2  "GPIO1/ENC0B/Fr0St/Ch0St"
  Manual Switch2/1 -> Mux1/3  "GPIO2/ENC0I/Fr0I/Ch0StSt  /  PWMO/ENC0I/Fr0I/Ch0StSt"
  Manual Switch3/1 -> Mux1/4  "GPIO3/ENC1A/Fr1G/Ch1G"
  Manual Switch4/1 -> Mux1/5  "GPIO4/ENC1B/Fr1St/Ch1St"
  Manual Switch5/1 -> Mux1/6  "GPIO5/ENC1I/Fr1I/Ch1StSt  /  PWM1/ENC1I/Fr1I/Ch1StSt"
  Manual Switch6/1 -> Mux1/7  "GPIO6/ENC2A/Fr2G/Ch2G"
  Manual Switch7/1 -> Mux1/8  "GPIO7/ENC2B/Fr2St/Ch2St"
  Manual Switch8/1 -> Mux1/9  "GPIO8/ENC2I/Fr2I/Ch2StSt  /  PWM2/ENC2I/Fr2I/Ch2StSt"
  Manual Switch9/1 -> Mux1/10  "GPIO9/ENC3A/Fr3G/Ch3G"
  Manual Switch10/1 -> Mux1/11  "GPIO10/ENC3B/Fr3St/Ch3St"
  Manual Switch11/1 -> Mux1/12  "GPIO11/ENC3I/Fr3I/Ch3StSt  /  PWM3/ENC3I/Fr3I/Ch3StSt"
  Manual Switch12/1 -> Mux1/13  "GPIO12/ENC4A/Fr4G/Ch4G"
  Manual Switch13/1 -> Mux1/14  "GPIO13/ENC4B/Fr4St/Ch4St"
  Manual Switch14/1 -> Mux1/15  "GPIO14/ENC4I/Fr4I/Ch4StSt  /  PWM4/ENC4I/Fr4I/Ch4StSt"
  Manual Switch15/1 -> Mux1/16  "GPIO15/ENC5A/Fr5G/Ch5G"
  Manual Switch16/1 -> Mux1/17  "GPIO16/ENC5B/Fr5St/Ch5St"
  Manual Switch17/1 -> Mux1/18  "GPIO17/ENC5I/Fr5I/Ch5StSt  /  PWM5/ENC5I/Fr5I/Ch5StSt"
  Manual Switch18/1 -> Mux1/19  "GPIO18/ENC6A/Fr6G/Ch6G"
  Manual Switch19/1 -> Mux1/20  "GPIO19/ENC6B/Fr6St/Ch6St"
  Manual Switch20/1 -> Mux1/21  "GPIO20/ENC6I/Fr6I/Ch6StSt  /  PWM6/ENC6I/Fr6I/Ch6StSt"
  Manual Switch21/1 -> Mux1/22  "GPIO21/ENC7A/Fr7G/Ch7G"
  Manual Switch22/1 -> Mux1/23  "GPIO22/ENC7B/Fr7St/Ch7St"
  Manual Switch23/1 -> Mux1/24  "GPIO23/ENC7I/Fr7I/Ch7StSt  /  PWM7/ENC7I/Fr7I/Ch7StSt"
  Manual Switch24/1 -> Mux1/25  "GPIO24/CNT0"
  Manual Switch25/1 -> Mux1/26  "GPIO25/CNT1"
  Mux1/1 -> For Subsystem/1(U)
  For Subsystem/1(Y) -> Data Type Conversion6/1, [SetCN1PinMode]
  Data Type Conversion6/1 -> Display/1

== system my_cascade_ramp116_rt/Magnetic Levitation System 1EM USB2/CN1 Digital I//O/Subsystem/For Subsystem ==
  U : Inport
  Assignment : Assignment  IndexOptions=Index vector (port)  Indices=1  OutputSizes=[([1 1])]
  Divide : Product
  Fcn : Fcn  Expr=2^(u-1)
  For Iterator : ForIterator  ResetStates=reset  IterationLimit=26  IterationVariableDataType=double
  Gain : Gain  Gain=ones(1,26)  Multiplication=Matrix(K*u)
  Selector : Selector  IndexOptions=Index vector (port)  Indices=[1 3]  OutputSizes=[(-2)]
  Y : Outport  VectorParamsAs1DForOutWhenUnconnected=off
  wires:
  Divide/1 -> Assignment/2
  Selector/1 -> Divide/1
  U/1 -> Selector/1, Assignment/1
  For Iterator/1 -> Selector/2, Fcn/1, Assignment/3
  Fcn/1 -> Divide/2
  Assignment/1 -> Gain/1
  Gain/1 -> Y/1

== system my_cascade_ramp116_rt/Magnetic Levitation System 1EM USB2/CN1 Digital I//O/Subsystem1/For Subsystem ==
  U : Inport
  Assignment : Assignment  IndexOptions=Index vector (port)  Indices=1  OutputSizes=[([1 1])]
  Divide : Product
  Fcn : Fcn  Expr=2^(u-1)
  For Iterator : ForIterator  ResetStates=reset  IterationLimit=26  IterationVariableDataType=double
  Gain : Gain  Gain=ones(1,26)  Multiplication=Matrix(K*u)
  Selector : Selector  IndexOptions=Index vector (port)  Indices=[1 3]  OutputSizes=[(-2)]
  Y : Outport  VectorParamsAs1DForOutWhenUnconnected=off
  wires:
  Gain/1 -> Y/1
  Assignment/1 -> Gain/1
  Fcn/1 -> Divide/2
  For Iterator/1 -> Assignment/3, Fcn/1, Selector/2
  U/1 -> Assignment/1, Selector/1
  Selector/1 -> Divide/1
  Divide/1 -> Assignment/2

== system my_cascade_ramp116_rt/Magnetic Levitation System 1EM USB2/CN1 Digital I//O/Subsystem2/For Subsystem ==
  U : Inport
  Assignment : Assignment  IndexOptions=Index vector (port)  Indices=1  OutputSizes=[([1 1])]
  Divide : Product
  Fcn : Fcn  Expr=2^(u-1)
  For Iterator : ForIterator  ResetStates=reset  IterationLimit=26  IterationVariableDataType=double
  Gain : Gain  Gain=ones(1,26)  Multiplication=Matrix(K*u)
  Selector : Selector  IndexOptions=Index vector (port)  Indices=[1 3]  OutputSizes=[(-2)]
  Y : Outport  VectorParamsAs1DForOutWhenUnconnected=off
  wires:
  Divide/1 -> Assignment/2
  Selector/1 -> Divide/1
  U/1 -> Selector/1, Assignment/1
  For Iterator/1 -> Selector/2, Fcn/1, Assignment/3
  Fcn/1 -> Divide/2
  Assignment/1 -> Gain/1
  Gain/1 -> Y/1
